simulink model "Lead"  (R2022a)
settings: Solver=VariableStepAuto  StartTime=0.0  StopTime=10.0  RelTol=1e-3
settings Model: Creator=user  LastModifiedBy=user

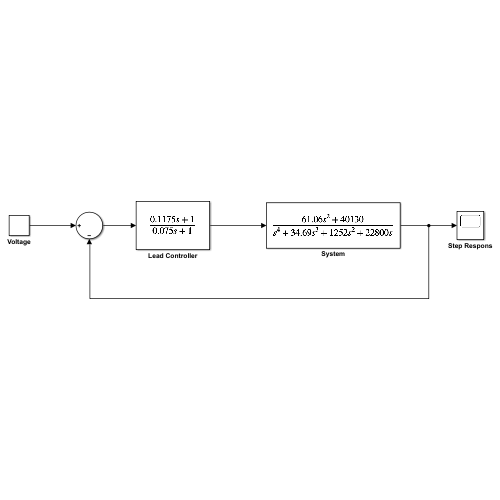
[thumbnail: Simulink's stored preview of the top-level diagram]
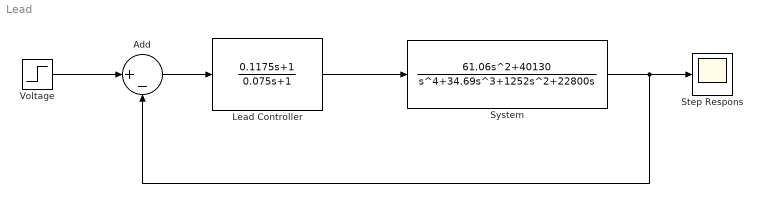
== system Lead ==
  Add : Sum  Inputs=|+-
  Lead Controller : TransferFcn  Numerator=[0.1175 1]  Denominator=[0.075 1]
  Step Respons : Scope
  System : TransferFcn  Numerator=[61.06 0 40130]  Denominator=[1 34.69 1252 22800 0]
  Voltage : Step  Time=0  SampleTime=0
  wires:
  System/1 -> Add/2, Step Respons/1
  Lead Controller/1 -> System/1
  Voltage/1 -> Add/1
  Add/1 -> Lead Controller/1
